simulink model "Horizontal1804"  (R2026b)
settings: Solver=FixedStepDiscrete  StopTime=inf  FixedStep=Official.Step
PostLoadFcn:
  | run(fullfile(fileparts(get_param('StampFly_IMU400','FileName')),'config','startup.m'));
InitFcn:
  | init_imu_flight;
undefined symbols (not defined in the file): Official
libraries: slpidlib x7, simulink x4, mspfiltlib x1
(part 5 of 5)

== matlab function Horizontal1804/FlightControl/TakeoffHoverControl/FlightCommand/ControlGating/ControlEnableReset ==
  data: arg_arg_raw input single; arg_arg_command output single; arg_arg_manual input boolean; arg_arg_auto input boolean; arg_branch input uint8; arg_arg_controlMode input single; arg_arg_dt input single; arg_arg_oldFilter input single; arg_arg_lastThrust input single; arg_arg_mode input uint8; arg_arg_run output boolean; arg_arg_reset output boolean; arg_arg_altEnable output boolean; arg_arg_angleEnable output boolean; arg_arg_velEnable output boolean
function [arg_arg_command,arg_arg_run,arg_arg_reset,arg_arg_altEnable,arg_arg_angleEnable,arg_arg_velEnable]=stepFn(arg_arg_raw,arg_arg_manual,arg_arg_auto,arg_branch,arg_arg_controlMode,arg_arg_dt,arg_arg_oldFilter,arg_arg_lastThrust,arg_arg_mode)
% 概要：共通推力指令の平滑化と各 PID の実行・リセット条件を決めます。推力を 3.7 V 基準の Duty に換算し、0.1 未満なら PID をリセットします。高度・角度・速度ループは操縦モードに応じて個別に有効にします。
%#codegen
% 1. 手動推力を 10 ms で平滑化し、指定された分岐では前回推力を保持します。
arg_arg_command=arg_arg_raw;
if arg_arg_manual,arg_arg_command=filterStep(arg_arg_raw,arg_arg_dt,single(.01),arg_arg_oldFilter);end
if arg_branch==5 || arg_branch==3,arg_arg_command=arg_arg_lastThrust;end
% 2. 通常飛行と着陸の有効分岐、および低推力のリセット条件を判定します。
active=arg_branch==2 || arg_branch==5;
arg_arg_reset=active && double(arg_arg_command)/3.7<double(single(.1));
arg_arg_run=active && ~arg_arg_reset;
% 3. Auto 高度、Stabilize 角度、鉛直速度の各ループの許可を分けて出力します。
arg_arg_altEnable=arg_arg_run && arg_arg_auto;
arg_arg_angleEnable=arg_arg_run && uint8(arg_arg_controlMode)==0;
arg_arg_velEnable=arg_arg_run && (arg_arg_auto || arg_arg_mode==5);
end
% 4. 局所関数：入力と前回値を dt・時定数で混合する一次低域フィルターです。
function s=filterStep(u,h,T,s),s=s*T/(T+h)+u*h/(T+h);end

== matlab function Horizontal1804/SensorCorrection/IMUBiasCalibration ==
  data: a input single; offset output single; g input single; mode input uint8; count output uint16
function [offset,count]=stepFn(a,g,mode)
% 概要：起動時に静止した機体のジャイロ XYZ と加速度 Z を 800 周期平均します。出力 Offset は [GyroX; GyroY; GyroZ; AccelZ]、Count は取得数です。400 Hz で公称 2 秒の校正中は機体を動かさないでください。
%#codegen
% 1. 平均値とサンプル数を初期化して保持します。
persistent Offset Count;
if isempty(Offset)
Offset=zeros(4,1,'single');
Count=uint16(0);
end
% 2. Mode 0 で初期化し、Mode 1 で 800 周期まで逐次平均を更新します。Mode 2 以降は校正値を保持します。
            if mode==0,Offset(:)=single(0);Count=uint16(0);
            elseif mode==1 && Count<uint16(800)
                n=single(Count);
                Offset=(n*Offset+[g;a(3)])/(n+single(1));
                Count=Count+uint16(1);
            end
% 3. 校正値の順序を維持し、フィルターと診断へ渡します。
            offset=Offset;count=Count;
end

== matlab function Horizontal1804/SensorCorrection/ToFHoldOutlierFilter ==
  data: mm input int16; alt output single; fresh input uint8; mode input uint8; dt input single; raw output int16
function [alt,raw]=stepFn(mm,fresh,mode,dt)
% 概要：新しい下向き距離 [mm] を保持・外れ値処理して高さ [m] へ変換します。20 mm 以下は前回の有効距離を使い、500 mm 超の飛びは最大 2 回まで履歴から補外します。Mode 0, 1 では推定用の出力を保持します。
%#codegen
% 1. 距離履歴、有効距離、生距離、外れ値回数、平滑化高さ、前回モードを保持します。
persistent History Range Raw Outlier Alt PreviousMode;
if isempty(History)
History=zeros(4,1,'int16');
Range=int16(0);
Raw=int16(0);
Outlier=uint8(0);
Alt=single(0);
PreviousMode=uint8(0);
end
% 2. 待機への移行時に履歴と平滑化高さを初期化します。
            if mode==3 && mode~=PreviousMode,History(:)=int16(0);Alt=single(0);end
% 3. 有効モードでのみ推定用の値を更新します。センサー自体の常時取得とは独立した条件です。
            if mode>1
% 4. Fresh の周期だけ生距離を受け取り、20 mm 超なら保持距離を更新します。
                if fresh~=0
                    Raw=mm;if mm>int16(20),Range=mm;end
                    delta=int32(Range)-int32(History(2));
% 5. 500 mm 超の飛びを検出し、直近履歴による補外を最大 2 回行います。正常値は履歴へ追加します。
                    if abs(delta)>int32(500) && Outlier<uint8(2)
                        extrap=int32(History(2))+idivide(int32(History(2))-int32(History(4)),int32(2),'fix');
                        Range=int16(extrap);Outlier=Outlier+uint8(1);
                    else
                        Outlier=uint8(0);History(4)=History(3);History(3)=History(2);History(2)=Range;
                    end
                end
% 6. 保持距離を m に換算し、時定数 5 ms で毎周期平滑化します。
                Alt=filterStep(single(double(Range)/1000),dt,single(0.005),Alt);
            end
            alt=Alt;raw=Raw;PreviousMode=mode;
end

% 7. 局所関数：既存の一次低域フィルター。演算順序を維持して前回値を更新します。
function s = filterStep(u,h,T,s)
%#codegen
s = s*T/(T+h) + u*h/(T+h);
end

== matlab function Horizontal1804/AttitudeAltitudeEstimation/AltitudeKalman ==
  data: alt input single; height output single; az input single; mode input uint8; dt input single; parkingReset input boolean; velocity output single; bias output single
function [height,velocity,bias]=stepFn(alt,az,mode,dt,parkingReset)
% 概要：下向き ToF の保持・平滑化した高さと鉛直加速度から、高度 [m]・鉛直速度・加速度バイアスを推定します。状態は [速度; 高度; バイアス]。公式実装の single 演算順序とリセット動作を保つ MATLAB Function です。加速度入力は従来どおり g 基準の数値です。
%#codegen
% 1. 推定状態、初回更新のフラグ、前周期のモードを記憶します。
persistent State First PreviousMode;
if isempty(State)
State=kalmanInitial();
First=false;
PreviousMode=uint8(0);
end
% 2. 待機リセットは共分散と公開出力を初期化します。内部の推定 x は保持します。
            if parkingReset,[~,State]=kalmanStep(single(0),single(0),dt,true,State);end
% 3. 待機への移行と最初の有効周期では 1 周期更新を見送り、Mode 0, 1 では推定を保持します。
            if mode==3 && mode~=PreviousMode,First=false;end
            if mode>1
                if First,[~,State]=kalmanStep(alt,az,dt,false,State);else,First=true;end
            end
% 4. 状態の順序を変えず、高度・速度・バイアスを個別の出力端子へ渡します。
            velocity=State.output(1);height=State.output(2);bias=State.output(3);PreviousMode=mode;
end

% 5. 局所関数：1 周期の予測と観測更新。dt は実測周期で、観測は毎周期の最新保持 ToF 値です。
function [y,s] = kalmanStep(z,acc,h,resetState,s)
%#codegen
% 6. リセット時は P=100I と公開出力 0。通常時は速度・高度・減衰するバイアスを予測します。
if resetState
    s.P = single(100)*eye(3,'single'); s.output(:) = single(0);
else
    p=s.P; b=single(-0.01); f=single(1)+h*b;
    xp=[s.x(1)+(acc-s.x(3))*h;s.x(2)+s.x(1)*h;s.x(3)*f];
% 7. 予測共分散を要素ごとに更新します。加速度雑音とバイアス変動の既存係数を使用します。
    pp=zeros(3,3,'single');
    pp(1,1)=p(1,1)-h*(p(3,1)+p(1,3))+h*h*p(3,3)+h*h*single(0.01);
    pp(1,2)=h*(p(1,1)-p(3,2))-h*h*p(3,1)+p(1,2);
    pp(1,3)=f*(p(1,3)-h*p(3,3));
    pp(2,1)=h*(p(1,1)-p(2,3))-h*h*p(1,3)+p(2,1);
    pp(2,2)=h*h*p(1,1)+h*(p(2,1)+p(1,2))+p(2,2);
    pp(2,3)=f*(p(2,3)+h*p(1,3));
    pp(3,1)=f*(p(3,1)-h*p(3,3));
    pp(3,2)=f*(p(3,2)+h*p(3,1));
    pp(3,3)=f*f*p(3,3)+h*h;
% 8. 高さの残差から Kalman ゲインで補正します。観測分散は (0.004 m)²。減算型の共分散更新も従来どおりです。
    k=[pp(1,2);pp(2,2);pp(3,2)]/(pp(2,2)+single(0.004*0.004));
    e=z-xp(2); s.x=xp+k*e; s.output=s.x;
    s.P(1,:)=pp(1,:)-k(1)*pp(2,:);
    s.P(2,:)=pp(2,:)*(single(1)-k(2));
    s.P(3,:)=-k(3)*pp(2,:)+pp(3,:);
end
y=s.output;
end

% 9. 局所関数：推定 x と公開出力を 0、初期共分散を 100I として生成します。
function s = kalmanInitial()
%#codegen
s = struct('x',zeros(3,1,'single'),'P',single(100)*eye(3,'single'), ...
    'output',zeros(3,1,'single'));
end

== matlab function Horizontal1804/AttitudeAltitudeEstimation/SensorFlags ==
  data: arg_accel input single; arg_flags output uint8; arg_azd input single; arg_voltage input single; arg_mode input uint8; arg_altFlag input uint8; arg_height input single; arg_rawRange input int16; arg_dt input single; arg_parkingReset input boolean
function arg_flags =stepFn(arg_accel,arg_azd,arg_voltage,arg_mode,arg_altFlag,arg_height,arg_rawRange,arg_dt,arg_parkingReset)
% 概要：推定・状態管理で使う [過大加速度; 距離異常の継続回数; 低電圧の継続回数] を uint8 で出力します。短い揺れを平滑化し、距離は最大 20 回、低電圧は最大 100 回まで数えます。
%#codegen
% 1. 加速度ノルムと電圧のフィルター状態、異常フラグ、前回モードを保持します。
persistent Norm Voltage OverG RangeFlag LowVoltage PreviousMode;
if isempty(Norm)
Norm=single(0);
Voltage=single(0);
OverG=uint8(0);
RangeFlag=uint8(0);
LowVoltage=uint8(0);
PreviousMode=uint8(0);
end
% 2. 待機リセットで過大加速度・距離異常を解除します。低電圧は 100 回到達後に保持します。
            if arg_parkingReset,OverG=uint8(0);RangeFlag=uint8(0);end
            if arg_mode==3 && arg_mode~=PreviousMode,Norm=single(0);end
% 3. 有効モードで、高度制御時の 2 m 超過または生距離 0 の継続を数えます。
            if arg_mode>1
                if (arg_height>single(2) && arg_altFlag~=0) || arg_rawRange==0,RangeFlag=min(RangeFlag+uint8(1),uint8(20));else,RangeFlag=uint8(0);end
            end
% 4. XY 加速度と校正後 Z 差分のノルムを 5 ms で平滑化し、2 g 超過をラッチします。
            normA=sqrt(arg_accel(1)*arg_accel(1)+arg_accel(2)*arg_accel(2)+arg_azd*arg_azd);
            Norm=filterStep(normA,arg_dt,single(.005),Norm);
            if Norm>single(2),OverG=uint8(1);end
% 5. 電圧を 5 ms で平滑化し、3.34 V 未満の連続回数を判定します。
            Voltage=filterStep(arg_voltage,arg_dt,single(.005),Voltage);
            if LowVoltage~=uint8(100)
                if Voltage<single(3.34),LowVoltage=LowVoltage+uint8(1);else,LowVoltage=uint8(0);end
                LowVoltage=min(LowVoltage,uint8(100));
            end
% 6. 既存のフラグ順序で公開し、次周期用にモードを保存します。
            arg_flags=[OverG;RangeFlag;LowVoltage];PreviousMode=arg_mode;
end

% 7. 局所関数：既存の一次低域フィルター。掛け算・割り算・加算の順序を維持します。
function s = filterStep(u,h,T,s)
%#codegen
s = s*T/(T+h) + u*h/(T+h);
end

== stateflow chart Horizontal1804/OfficialFlightSupervisor ==
  settings: description=|
      | 飛行モードの状態遷移図（400 Hz）
      | INIT→AVERAGE→PARKING→FLIGHT→LANDING。通信途絶・OverG・ボタンを遷移条件で判断。
      | CycleInputsが1周期分の入力を整理し、syncで前周期の確定状態に同期、decideで今回の遷移を実行。
      | branchは今回の分岐開始状態、modeは今回の判断後の状態。MATLAB関数はChart内に置かない。
  state FlightModes [parallel]
    settings: executionOrder=1
    state PARKING
      en: mode=uint8(3);
    state AVERAGE
      en: mode=uint8(1);
    state INIT
      en: mode=uint8(0);
    state FLIGHT
      en: mode=uint8(2);
    state LANDING
      en: mode=uint8(5);
    state OTHER
      en: mode=branch;
    (default) -> INIT : /{calibration=uint16(0); buttonCounter=int8(0); buttonState=uint8(0); chatter=uint8(0); lastAHRS=uint8(0); connectionCounter=uint16(0); buttonEvent=false; calibrationDone=false;}
    AVERAGE -> PARKING : decide[calibrationDone]
    INIT -> AVERAGE : decide
    (junction 43) -> AVERAGE [order 2] : [branch==uint8(1)]
    (junction 43) -> INIT [order 1] : [branch==uint8(0)]
    PARKING -> FLIGHT : decide[buttonEvent]/{ahrsReset=true;}
    FLIGHT -> PARKING [order 1] : decide[flags(1)==1]/{ahrsReset=true;}
    (junction 43) -> PARKING [order 3] : [branch==uint8(3)]
    LANDING -> PARKING : decide[buttonEvent]
    FLIGHT -> LANDING [order 2] : decide[buttonEvent || connected==0]/{ahrsReset=true;}
    (junction 43) -> LANDING [order 5] : [branch==uint8(5)]
    (junction 43) -> FLIGHT [order 4] : [branch==uint8(2)]
    FlightModes -> (junction 43) : sync
    (junction 43) -> OTHER [order 6]
  state CycleInputs [parallel]
    en: branch=previousMode; mode=branch; ahrsReset=false; parkingReset=branch==3;
    buttonEvent=false; calibrationDone=false;
    if newPacket~=0, connectionCounter=uint16(0); end
    connected=uint8(connectionCounter<uint16(40));
    if branch==1
    calibrationDone=calibration>=uint16(800);
    if ~calibrationDone, calibration=calibration+uint16(1); end
    elseif branch~=0
    if button==1
    buttonCounter=buttonCounter+int8(1);
    if buttonCounter>int8(10),buttonCounter=int8(10);buttonState=uint8(1);end
    else
    buttonCounter=buttonCounter-int8(1);
    if buttonCounter<int8(-10),buttonCounter=int8(-10);buttonState=uint8(0);end
    end
    if chatter==0
    if buttonState==1,chatter=uint8(1);end
    elseif buttonState==0
    chatter=chatter+uint8(1);
    if chatter>uint8(40),chatter=uint8(0);buttonEvent=true;end
    end
    if branch==3
    if ahrsFlag~=lastAHRS
    if ahrsFlag==1,ahrsReset=true;end
    lastAHRS=ahrsFlag;
    end
    elseif branch==2
    connectionCounter=uint16(mod(double(connectionCounter)+1,65536));
    connected=uint8(connectionCounter<uint16(40));
    end
    end
    send(sync,FlightModes);
    send(decide,FlightModes);
    du: branch=previousMode; mode=branch; ahrsReset=false; parkingReset=branch==3;
    buttonEvent=false; calibrationDone=false;
    if newPacket~=0, connectionCounter=uint16(0); end
    connected=uint8(connectionCounter<uint16(40));
    if branch==1
    calibrationDone=calibration>=uint16(800);
    if ~calibrationDone, calibration=calibration+uint16(1); end
    elseif branch~=0
    if button==1
    buttonCounter=buttonCounter+int8(1);
    if buttonCounter>int8(10),buttonCounter=int8(10);buttonState=uint8(1);end
    else
    buttonCounter=buttonCounter-int8(1);
    if buttonCounter<int8(-10),buttonCounter=int8(-10);buttonState=uint8(0);end
    end
    if chatter==0
    if buttonState==1,chatter=uint8(1);end
    elseif buttonState==0
    chatter=chatter+uint8(1);
    if chatter>uint8(40),chatter=uint8(0);buttonEvent=true;end
    end
    if branch==3
    if ahrsFlag~=lastAHRS
    if ahrsFlag==1,ahrsReset=true;end
    lastAHRS=ahrsFlag;
    end
    elseif branch==2
    connectionCounter=uint16(mod(double(connectionCounter)+1,65536));
    connected=uint8(connectionCounter<uint16(40));
    end
    end
    send(sync,FlightModes);
    send(decide,FlightModes);
    settings: executionOrder=2
  note: 飛行モードの状態遷移図（400 Hz）
      | INIT→AVERAGE→PARKING→FLIGHT→LANDING。通信途絶・OverG・ボタンを遷移条件で判断。
      | CycleInputsが1周期分の入力を整理し、syncで前周期の確定状態に同期、decideで今回の遷移を実行。
      | branchは今回の分岐開始状態、modeは今回の判断後の状態。MATLAB関数はChart内に置かない。
  data: previousMode input uint8; button input uint8; newPacket input uint8; flags input uint8; ahrsFlag input uint8; branch output uint8; mode output uint8; ahrsReset output boolean; parkingReset output boolean; connected output uint8; calibration local uint16; buttonCounter local int8; buttonState local uint8; chatter local uint8; lastAHRS local uint8; connectionCounter local uint16; buttonEvent local boolean; calibrationDone local boolean
  events: sync local FUNCTION_CALL_EVENT; decide local FUNCTION_CALL_EVENT
